simulink model "dx300_boom_hyd"  (R2026b)
settings: Solver=daessc  StopTime=10  AbsTol=1e-3  EnableMultiTasking=on
InitFcn:
  | here='/home/ahmed/ahmed/dx300-sim/matlab/lab08a'; run(fullfile(here,'dx300_params_lab08a.m')); load(fullfile(here,'stage2_mass.mat')); J_cm = P.m_boom*P.L_boom^2/12; La=3.1; phi_rel=deg2rad(-90); m_Dpt=340; m_armpt=1050+220; m_tippt=1120+1.27*1800;
  | S1 = load(fullfile(here,'stage1_kin.mat'),'th','r'); th_tab = S1.th(:)';  r_tab = S1.r(:)';  % moment arm r(theta), m (from ESTIMATED pins)
  | % --- Stage 4 hydraulics ---
  | A_cap = P.n_cyl*pi/4*P.bore^2;                 % OFFICIAL-derived [m^2] combined cap area of 2 cylinders
  | A_ann = P.n_cyl*pi/4*(P.bore^2-P.rod^2);       % OFFICIAL-derived [m^2] combined annulus area
  | rho_oil = 870;      % kg/m^3  ESTIMATED (typical mineral hydraulic oil)
  | beta_oil = 1.5e9;   % Pa      ESTIMATED (typical effective bulk modulus)
  | nu_oil = 46e-6;     % m^2/s   ESTIMATED (ISO VG46-ish, ~46 cSt)
  | A_valve_max = 3e-4; % m^2     ESTIMATED (main spool / relief max area)
  | dS_max = 5e-3;      % m       ESTIMATED (spool stroke)
  | p_range_relief = 5e5; % Pa    ESTIMATED (relief opening range)
  | V_dead = 1e-3;      % m^3     ESTIMATED (dead volume per chamber incl. hose/gallery, both cylinders)
  | % static holding pressure at th_min (analytic gravity torque as in stage3_validate) -> consistent initial cap pressure
  | q0_ = P.th_min; pts_ = [P.L_boom 0; P.L_boom+0.5*La*cos(phi_rel) 0.5*La*sin(phi_rel); P.L_boom+La*cos(phi_rel) La*sin(phi_rel)];
  | tau_g0 = P.m_boom*9.81*Lc0*cos(q0_) + 9.81*([m_Dpt m_armpt m_tippt]*(pts_(:,1)*cos(q0_)-pts_(:,2)*sin(q0_)));   % N m
  | p0_cap = tau_g0/(r_tab(1)*A_cap) + 101325;   % Pa abs
  | spool_t = 1.0;      % s       spool step time (design choice)
values from neighbouring files (symbols this model uses):
  m = dst    [build_stage4.m]    (also in stage2_mass.m = P.m_boom; stage3_validate.m = 'dx300_boom_mb'; stage4_run.m = 'dx300_boom_hyd')
  N = 2^nextpow2(4*numel(pd))    [stage5_damping.m]
  s = get_param([m '/theta_cmd'],'PortHandles')    [stage3_validate.m]    (also in stage4_run.m = Ft.Time > 3)
  Y = abs(fft(pd.*hann(numel(pd)), N))    [stage5_damping.m]
undefined symbols (not defined in the file or in its folder): P, X, Z
libraries: fl_lib x16, nesl_utility x12, sm_lib x11, SimscapeFluids_lib x3, simulink x1
settings Model: Creator=ahmed  LastModifiedBy=ahmed
settings SolverCC: AutoScaleAbsTol=off
settings DataIOCC: LimitDataPoints=on  MaxDataPoints=10000
settings OptimizationCC: LifeSpan=inf  ReuseModelBlockBuffer=off
settings DebuggingCC: AllowSymbolicDim=off  ArithmeticOperatorsInVariantConditions=warning  SFExecutionAtInitializationDiag=none  SFNoUnconditionalDefaultTransitionDiag=warning  SFUnexpectedBacktrackingDiag=warning  SubsystemReferenceDiagnosticForUnitTest=warning
settings SFSimCC: CustomCodeUndefinedFunction=UseInterfaceOnly  SimUseLocalCustomCode=off
settings RTWCC: DLArmComputeVersion=19.05  RTWUseLocalCustomCode=off
settings CodeAppCC: StateflowObjectComments=on
settings GRTTargetCC: TargetLangStandard=C89/C90 (ANSI)
settings ConfigComp: CovExternalEMLEnable=off  CovSFcnEnable=off  CovSaveCumulativeToWorkspaceVar=on  CovSaveSingleToWorkspaceVar=on
settings SimscapeCC: SimscapeLogType=all  SimscapeUseEnergyAccounting=off

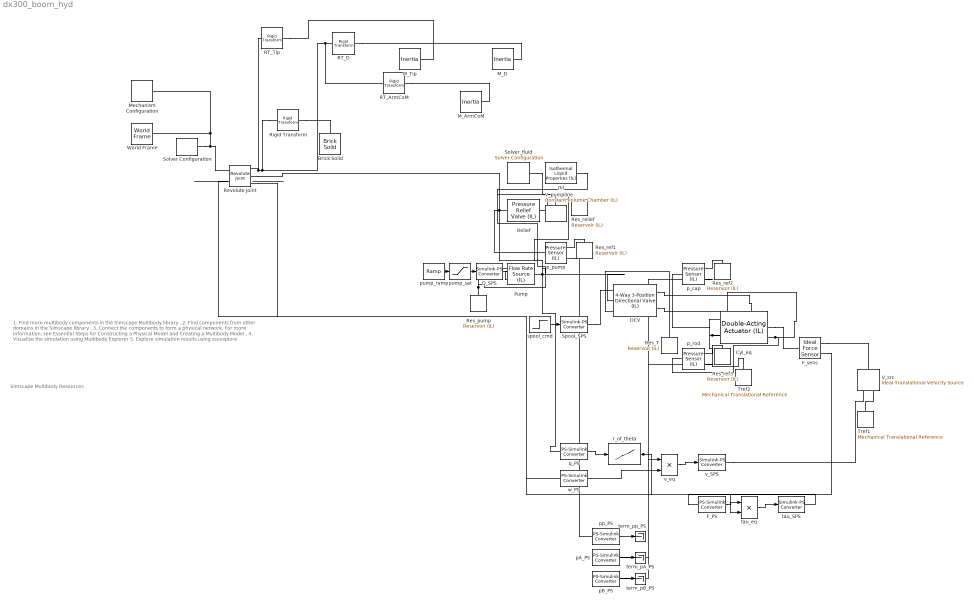
== system dx300_boom_hyd ==
  note: 1. Find more multibody components in the Simscape Multibody library .
      | 2. Find components from other domains in the Simscape library .
      | 3. Connect the components to form a physical network.
      | For more information, see Essential Steps for Constructing a Physical Model and Creating a Multibody Model .
      | 4. Visualize the simulation using Multibody Explorer
      | 5. Explore simulation results using sscexplore
  note: Simscape Multibody Resources
  Brick Solid : sm_lib/Body Elements/Brick Solid  BrickDimensions=[P.L_boom 0.5 0.5]  BrickDimensionsUnits=m  ExportEntireGeometry=off  InertiaType=CalculateFromGeometry  BasedOnType=Mass  Density=1000  DensityUnits=kg/m^3  Mass=2330  MassUnits=kg  CenterOfMass=[0 0 0]  CenterOfMassUnits=m  MomentsOfInertia=[1 1 1]  MomentsOfInertiaUnits=kg*m^2  ProductsOfInertia=[0 0 0]  ProductsOfInertiaUnits=kg*m^2  GraphicType=FromGeometry  MarkerShape=Sphere  MarkerSize=10  GraphicVisPropType=SimpleVisualProperties  GraphicDiffuseColor=[0.5 0.5 0.5]  GraphicOpacity=1.0  GraphicSpecularColor=[0.5 0.5 0.5 1.0]  GraphicAmbientColor=[0.15 0.15 0.15 1.0]  GraphicEmissiveColor=[0.0 0.0 0.0 1.0]  GraphicShininess=75  DoExposeReferenceFrame=on  SerializedFrames=<Frames/>
  Cyl_eq : SimscapeFluids_lib/Isothermal Liquid/Actuators/Double-Acting Actuator (IL)  single_fluid=true  mech_orientation=foundation.enum.MechOrientationTranslational.Positive  piston_area_A=A_cap m^2  piston_area_B=A_ann m^2  stroke=P.stroke m  dead_volume_A=V_dead m^3  dead_volume_B=V_dead m^3  pressure_spec=foundation.enum.pressure_spec.atmospheric  environment_pressure=0.101325 MPa  hardstop_model=simscape.enum.hardstop.smooth  stiff_coeff=1e10 N/m  damping_coeff=150 N*s/m  transition=0.1 mm  coeff_rest=0.7  v_tol=0.001 m/s  f_tol=0.001 N  cushion_A_spec=false  area_plunger_A=1e-4 m^2  length_plunger_A=1e-3 m  area_cushion_orifice_A=1e-6 m^2  area_leak_plunger_A=1e-7 m^2  p_crack_differential_A=0.01 MPa  press_max_differential_A=0.1 MPa  check_valve_area_max_A=1e-4 m^2  check_valve_area_leak_A=1e-10 m^2  smoothing_factor_A=0.01  cushion_B_spec=false  area_plunger_B=1e-4 m^2  length_plunger_B=1e-3 m  area_cushion_orifice_B=1e-6 m^2  area_leak_plunger_B=1e-7 m^2  p_crack_differential_B=0.01 MPa  press_max_differential_B=0.1 MPa  check_valve_area_max_B=1e-4 m^2  check_valve_area_leak_B=1e-10 m^2  smoothing_factor_B=0.01  friction_spec=false  breakaway_Coulomb_ratio=1.2  breakaway_velocity=0.1 m/s  preload_force=20 N  Coulomb_coeff=1e-6 N/Pa  viscous_coeff=100 N*s/m  leakage_spec=false  clearance=1e-4 m  piston_length=0.01 m  displacement_spec=foundation.enum.DisplacementSpec.Calculate  x0=0 m  dynamic_compressibility=true  p0_A=p0_cap Pa  p0_B=0.101325 MPa  p_nominal_A=0.101325 MPa  p_nominal_B=0.101325 MPa
  DCV : SimscapeFluids_lib/Isothermal Liquid/Valves & Orifices/Directional Control Valves/4-Way 3-Position Directional Valve (IL)  open_orifices_pos=fluids.isothermal_liquid.valves_orifices.directional_control_valves.enum.directional_valve_open_orifices_pos_neg.PA_BT  open_orifices_neu=fluids.isothermal_liquid.valves_orifices.directional_control_valves.enum.directional_valve_open_orifices_neutral.all_closed  open_orifices_neg=fluids.isothermal_liquid.valves_orifices.directional_control_valves.enum.directional_valve_open_orifices_pos_neg.PB_AT  neutral_assert_action=simscape.enum.assert.action.warn  area_spec=fluids.isothermal_liquid.valves_orifices.directional_control_valves.enum.directional_valve_area_spec.identical  valve_spec=fluids.isothermal_liquid.valves_orifices.directional_control_valves.enum.directional_valve_spec.linear  del_S_max=dS_max m  area_max=A_valve_max m^2  del_S_TLU=[0, .00125, .0025, .00375, .005] m  valve_area_TLU=[1e-10, 1e-05, 4e-05, 6e-05, .0001] m^2  del_S_vol_flow_TLU=[0, .00125, .0025, .00375, .005] m  p_diff_TLU=[-.1, .3, .5, .7] MPa  vol_flow_TLU=[-1e-08, 2.2e-08, 2.8e-08, 3.4e-08; -9e-06, .00015, .0002, .00024; -.00036, .00063, .00081, .00096; -.00054, .00094, .0012, .0014; -.00091, .0016, .002, .0024] m^3/s  p_diff_TLU_const=[-.1, .3, .5, .7] MPa  vol_flow_TLU_const=[-.0009, .0016, .002, .0024] m^3/s  area_const=1e-4 m^2  area_leak=1e-10 m^2  area=inf m^2  Cd=0.64  Re_c=150  smoothing_factor=0.01  pressure_recovery=false  S_max_PA=7.5e-3 m  del_S_max_PA=0.005 m  area_max_PA=1e-4 m^2  del_S_TLU_PA=[0, .00125, .0025, .00375, .005] m  valve_area_TLU_PA=[1e-10, 1e-05, 4e-05, 6e-05, .0001] m^2  del_S_vol_flow_TLU_PA=[0, .00125, .0025, .00375, .005] m  p_diff_TLU_PA=[-.1, .3, .5, .7] MPa  vol_flow_TLU_PA=[-1e-08, 2.2e-08, 2.8e-08, 3.4e-08; -9e-06, .00015, .0002, .00024; -.00036, .00063, .00081, .00096; -.00054, .00094, .0012, .0014; -.00091, .0016, .002, .0024] m^3/s  area_const_PA=1e-4 m^2  p_diff_TLU_const_PA=[-.1, .3, .5, .7] MPa  vol_flow_TLU_const_PA=[-.0009, .0016, .002, .0024] m^3/s  S_max_PB=-7.5e-3 m  del_S_max_PB=0.005 m  area_max_PB=1e-4 m^2  del_S_TLU_PB=[0, .00125, .0025, .00375, .005] m  valve_area_TLU_PB=[1e-10, 1e-05, 4e-05, 6e-05, .0001] m^2  del_S_vol_flow_TLU_PB=[0, .00125, .0025, .00375, .005] m  p_diff_TLU_PB=[-.1, .3, .5, .7] MPa  vol_flow_TLU_PB=[-1e-08, 2.2e-08, 2.8e-08, 3.4e-08; -9e-06, .00015, .0002, .00024; -.00036, .00063, .00081, .00096; -.00054, .00094, .0012, .0014; -.00091, .0016, .002, .0024] m^3/s  area_const_PB=1e-4 m^2  p_diff_TLU_const_PB=[-.1, .3, .5, .7] MPa  vol_flow_TLU_const_PB=[-.0009, .0016, .002, .0024] m^3/s  S_max_AB=7.5e-3 m  del_S_max_AB=0.005 m  area_max_AB=1e-4 m^2  del_S_TLU_AB=[0, .00125, .0025, .00375, .005] m  valve_area_TLU_AB=[1e-10, 1e-05, 4e-05, 6e-05, .0001] m^2  del_S_vol_flow_TLU_AB=[0, .00125, .0025, .00375, .005] m  p_diff_TLU_AB=[-.1, .3, .5, .7] MPa  vol_flow_TLU_AB=[-1e-08, 2.2e-08, 2.8e-08, 3.4e-08; -9e-06, .00015, .0002, .00024; -.00036, .00063, .00081, .00096; -.00054, .00094, .0012, .0014; -.00091, .0016, .002, .0024] m^3/s  area_const_AB=1e-4 m^2  p_diff_TLU_const_AB=[-.1, .3, .5, .7] MPa  vol_flow_TLU_const_AB=[-.0009, .0016, .002, .0024] m^3/s  S_max_AT=-7.5e-3 m  del_S_max_AT=0.005 m  area_max_AT=1e-4 m^2  del_S_TLU_AT=[0, .00125, .0025, .00375, .005] m  valve_area_TLU_AT=[1e-10, 1e-05, 4e-05, 6e-05, .0001] m^2  del_S_vol_flow_TLU_AT=[0, .00125, .0025, .00375, .005] m  p_diff_TLU_AT=[-.1, .3, .5, .7] MPa  vol_flow_TLU_AT=[-1e-08, 2.2e-08, 2.8e-08, 3.4e-08; -9e-06, .00015, .0002, .00024; -.00036, .00063, .00081, .00096; -.00054, .00094, .0012, .0014; -.00091, .0016, .002, .0024] m^3/s  area_const_AT=1e-4 m^2  p_diff_TLU_const_AT=[-.1, .3, .5, .7] MPa  vol_flow_TLU_const_AT=[-.0009, .0016, .002, .0024] m^3/s  S_max_BT=7.5e-3 m  del_S_max_BT=0.005 m  area_max_BT=1e-4 m^2  del_S_TLU_BT=[0, .00125, .0025, .00375, .005] m  valve_area_TLU_BT=[1e-10, 1e-05, 4e-05, 6e-05, .0001] m^2  del_S_vol_flow_TLU_BT=[0, .00125, .0025, .00375, .005] m  p_diff_TLU_BT=[-.1, .3, .5, .7] MPa  vol_flow_TLU_BT=[-1e-08, 2.2e-08, 2.8e-08, 3.4e-08; -9e-06, .00015, .0002, .00024; -.00036, .00063, .00081, .00096; -.00054, .00094, .0012, .0014; -.00091, .0016, .002, .0024] m^3/s  area_const_BT=1e-4 m^2  p_diff_TLU_const_BT=[-.1, .3, .5, .7] MPa  vol_flow_TLU_const_BT=[-.0009, .0016, .002, .0024] m^3/s  S_max_PT=0 m  del_S_max_PT=0.005 m  area_max_PT=1e-4 m^2  del_S_TLU_PT=[0, .00125, .0025, .00375, .005] m  valve_area_TLU_PT=[1e-10, 1e-05, 4e-05, 6e-05, .0001] m^2  del_S_vol_flow_TLU_PT=[0, .00125, .0025, .00375, .005] m  p_diff_TLU_PT=[-.1, .3, .5, .7] MPa  vol_flow_TLU_PT=[-1e-08, 2.2e-08, 2.8e-08, 3.4e-08; -9e-06, .00015, .0002, .00024; -.00036, .00063, .00081, .00096; -.00054, .00094, .0012, .0014; -.00091, .0016, .002, .0024] m^3/s
  F_PS : nesl_utility/PS-Simulink Converter  PhysicalDomain=network_engine_domain  SubClassName=ps_output  LeftPortType=input  RightPortType=output  PseudoPeriodic=off  Frequencies=[]  VectorFormat=inherit  Unit=N  AffineConversion=off
  F_sens : fl_lib/Mechanical/Mechanical Sensors/Ideal Force Sensor
  M_ArmCoM : sm_lib/Body Elements/Inertia  InertiaType=PointMass  Mass=m_armpt  MassUnits=kg  CenterOfMass=[0 0 0]  CenterOfMassUnits=m  MomentsOfInertia=[1 1 1]  MomentsOfInertiaUnits=kg*m^2  ProductsOfInertia=[0 0 0]  ProductsOfInertiaUnits=kg*m^2  GraphicType=Marker  MarkerShape=Inertia  MarkerSize=20  GraphicVisPropType=SimpleVisualProperties  GraphicDiffuseColor=[0.5 0.5 0.5]  GraphicOpacity=1  GraphicSpecularColor=[0.5 0.5 0.5 1.0]  GraphicAmbientColor=[0.15 0.15 0.15 1.0]  GraphicEmissiveColor=[0.0 0.0 0.0 1.0]  GraphicShininess=75
  M_D : sm_lib/Body Elements/Inertia  InertiaType=PointMass  Mass=m_Dpt  MassUnits=kg  CenterOfMass=[0 0 0]  CenterOfMassUnits=m  MomentsOfInertia=[1 1 1]  MomentsOfInertiaUnits=kg*m^2  ProductsOfInertia=[0 0 0]  ProductsOfInertiaUnits=kg*m^2  GraphicType=Marker  MarkerShape=Inertia  MarkerSize=20  GraphicVisPropType=SimpleVisualProperties  GraphicDiffuseColor=[0.5 0.5 0.5]  GraphicOpacity=1  GraphicSpecularColor=[0.5 0.5 0.5 1.0]  GraphicAmbientColor=[0.15 0.15 0.15 1.0]  GraphicEmissiveColor=[0.0 0.0 0.0 1.0]  GraphicShininess=75
  M_Tip : sm_lib/Body Elements/Inertia  InertiaType=PointMass  Mass=m_tippt  MassUnits=kg  CenterOfMass=[0 0 0]  CenterOfMassUnits=m  MomentsOfInertia=[1 1 1]  MomentsOfInertiaUnits=kg*m^2  ProductsOfInertia=[0 0 0]  ProductsOfInertiaUnits=kg*m^2  GraphicType=Marker  MarkerShape=Inertia  MarkerSize=20  GraphicVisPropType=SimpleVisualProperties  GraphicDiffuseColor=[0.5 0.5 0.5]  GraphicOpacity=1  GraphicSpecularColor=[0.5 0.5 0.5 1.0]  GraphicAmbientColor=[0.15 0.15 0.15 1.0]  GraphicEmissiveColor=[0.0 0.0 0.0 1.0]  GraphicShininess=75
  Mechanism Configuration : sm_lib/Utilities/Mechanism Configuration  UniformGravity=Constant  GravityVector=[0 -9.81 0]  GravityVectorUnits=m/s^2  LinearizationDelta=0.001  JointModeTransitionNonlinearIterations=2
  Oil : fl_lib/Isothermal Liquid/Utilities/Isothermal Liquid Properties (IL)  rho_L_atm=rho_oil kg/m^3  bulk_modulus_model=foundation.enum.bulk_modulus_model.const  beta_gain=6  beta_L_atm=beta_oil Pa  nu_atm=nu_oil m^2/s  p_atm=0.101325 MPa  p_min=1 Pa  properties_range_check=simscape.enum.assert.action.error  air_fraction=0.005  polytropic_index=1.0  rho_g_atm=1.225 kg/m^3  air_dissolution_model=false  p_crit=3 MPa
  Pump : fl_lib/Isothermal Liquid/Sources/Flow Rate Source (IL)  source_type=foundation.enum.constant_controlled.controlled  flow_type=foundation.enum.mass_volumetric_flow.volumetric  mass_flow=0 kg/s  volumetric_flow=0 m^3/s
  Q_SPS : nesl_utility/Simulink-PS Converter  PhysicalDomain=network_engine_domain  SubClassName=ps_input  LeftPortType=input  RightPortType=output  PseudoPeriodic=off  Frequencies=[]  NoiseDistribution=none  NoiseParameters=[]  Unit=m^3/s  AffineConversion=off  FilteringAndDerivatives=filter  SimscapeFilterOrder=2  InputFilterTimeConstant=0.001  UdotUserProvided=0
  RT_ArmCoM : sm_lib/Frames and Transforms/Rigid Transform  RotationMethod=None  FollAlignAxisA=+X  BaseAlignAxisA=+Y  FollAlignAxisB=+Y  BaseAlignAxisB=+Z  RotationStandardAxis=+Z  RotationAngle=0  RotationAngleUnits=deg  RotationArbitraryAxis=[0 0 1]  RotationSequenceAxes=FollowerAxes  RotationSequence=XYX  RotationSequenceAngles=[0 0 0]  RotationSequenceAnglesUnits=deg  RotationMatrix=[1 0 0;0 1 0;0 0 1]  Quaternion=[1 0 0 0]  TranslationMethod=Cartesian  TranslationCartesianOffset=[P.L_boom+0.5*La*cos(phi_rel) 0.5*La*sin(phi_rel) 0]  TranslationCartesianOffsetUnits=m  TranslationStandardAxis=+Z  TranslationStandardOffset=0  TranslationStandardOffsetUnits=m  TranslationROffset=0  TranslationROffsetUnits=m  TranslationThetaOffset=0  TranslationThetaOffsetUnits=deg  TranslationZOffset=0  TranslationZOffsetUnits=m
  RT_D : sm_lib/Frames and Transforms/Rigid Transform  RotationMethod=None  FollAlignAxisA=+X  BaseAlignAxisA=+Y  FollAlignAxisB=+Y  BaseAlignAxisB=+Z  RotationStandardAxis=+Z  RotationAngle=0  RotationAngleUnits=deg  RotationArbitraryAxis=[0 0 1]  RotationSequenceAxes=FollowerAxes  RotationSequence=XYX  RotationSequenceAngles=[0 0 0]  RotationSequenceAnglesUnits=deg  RotationMatrix=[1 0 0;0 1 0;0 0 1]  Quaternion=[1 0 0 0]  TranslationMethod=Cartesian  TranslationCartesianOffset=[P.L_boom 0 0]  TranslationCartesianOffsetUnits=m  TranslationStandardAxis=+Z  TranslationStandardOffset=0  TranslationStandardOffsetUnits=m  TranslationROffset=0  TranslationROffsetUnits=m  TranslationThetaOffset=0  TranslationThetaOffsetUnits=deg  TranslationZOffset=0  TranslationZOffsetUnits=m
  RT_Tip : sm_lib/Frames and Transforms/Rigid Transform  RotationMethod=None  FollAlignAxisA=+X  BaseAlignAxisA=+Y  FollAlignAxisB=+Y  BaseAlignAxisB=+Z  RotationStandardAxis=+Z  RotationAngle=0  RotationAngleUnits=deg  RotationArbitraryAxis=[0 0 1]  RotationSequenceAxes=FollowerAxes  RotationSequence=XYX  RotationSequenceAngles=[0 0 0]  RotationSequenceAnglesUnits=deg  RotationMatrix=[1 0 0;0 1 0;0 0 1]  Quaternion=[1 0 0 0]  TranslationMethod=Cartesian  TranslationCartesianOffset=[P.L_boom+La*cos(phi_rel) La*sin(phi_rel) 0]  TranslationCartesianOffsetUnits=m  TranslationStandardAxis=+Z  TranslationStandardOffset=0  TranslationStandardOffsetUnits=m  TranslationROffset=0  TranslationROffsetUnits=m  TranslationThetaOffset=0  TranslationThetaOffsetUnits=deg  TranslationZOffset=0  TranslationZOffsetUnits=m
  Relief : SimscapeFluids_lib/Isothermal Liquid/Valves & Orifices/Pressure Control Valves/Pressure Relief Valve (IL)  set_pressure_spec=foundation.enum.constant_controlled.constant  opening_spec=fluids.isothermal_liquid.valves_orifices.enum.PressureOpeningSpec.Linear  pressure_spec=fluids.isothermal_liquid.valves_orifices.enum.pressure_control_spec.pA  p_set_gauge=P.p_relief Pa  p_set_differential=0 MPa  p_range=p_range_relief Pa  area_max=A_valve_max m^2  area_leak=1e-10 m^2  p_diff_TLU=[0.2 : 0.2 : 1.2] MPa  p_gauge_TLU=[0.2 : 0.2 : 1.2] MPa  valve_area_TLU=[1e-10, 2e-06, 4e-06, 6e-06, 8e-06, 1e-05] m^2  vol_flow_TLU=[1e-09, 3.6e-05, 8.9e-05, .00015, .00023, .00031] m^3/s  area=inf m^2  Cd=0.64  Re_c=150  smoothing_factor=0.01  pressure_recovery=false  opening_dynamics=false  tau=0.1 s
  Res_T : fl_lib/Isothermal Liquid/Elements/Reservoir (IL)  pressure_input=false  pressure_spec=foundation.enum.pressure_spec.atmospheric  reservoir_pressure=0.101325 MPa
  Res_pump : fl_lib/Isothermal Liquid/Elements/Reservoir (IL)  pressure_input=false  pressure_spec=foundation.enum.pressure_spec.atmospheric  reservoir_pressure=0.101325 MPa
  Res_ref1 : fl_lib/Isothermal Liquid/Elements/Reservoir (IL)  pressure_input=false  pressure_spec=foundation.enum.pressure_spec.atmospheric  reservoir_pressure=0.101325 MPa
  Res_ref2 : fl_lib/Isothermal Liquid/Elements/Reservoir (IL)  pressure_input=false  pressure_spec=foundation.enum.pressure_spec.atmospheric  reservoir_pressure=0.101325 MPa
  Res_ref3 : fl_lib/Isothermal Liquid/Elements/Reservoir (IL)  pressure_input=false  pressure_spec=foundation.enum.pressure_spec.atmospheric  reservoir_pressure=0.101325 MPa
  Res_relief : fl_lib/Isothermal Liquid/Elements/Reservoir (IL)  pressure_input=false  pressure_spec=foundation.enum.pressure_spec.atmospheric  reservoir_pressure=0.101325 MPa
  Revolute Joint : sm_lib/Joints/Revolute Joint  JointMode=Normal  CompositeWrenchDir=FollowerOnBase  CompositeWrenchFrame=BaseFrame  SenseConstraintForce=off  SenseConstraintTorque=off  SenseTotalForce=off  SenseTotalTorque=off  PositionTargetSpecify=on  PositionTargetPriority=High  PositionTargetValue=P.th_min*180/pi  PositionTargetValueUnits=deg  VelocityTargetSpecify=off  VelocityTargetPriority=High  VelocityTargetValue=0  VelocityTargetValueUnits=deg/s  EquilibriumPosition=0  EquilibriumPositionUnits=deg  SpringStiffness=0  SpringStiffnessUnits=N*m/deg  DampingCoefficient=0  DampingCoefficientUnits=N*m/(deg/s)  LowerLimitSpecify=off  LowerLimitBound=-90  LowerLimitBoundUnits=deg  LowerLimitStiffness=1e4  LowerLimitStiffnessUnits=N*m/deg  LowerLimitDamping=10  LowerLimitDampingUnits=N*m/(deg/s)  LowerLimitTransitionRegionWidth=0.1  LowerLimitTransitionRegionWidthUnits=deg  UpperLimitSpecify=off  UpperLimitBound=90  UpperLimitBoundUnits=deg  UpperLimitStiffness=1e4  UpperLimitStiffnessUnits=N*m/deg  UpperLimitDamping=10  UpperLimitDampingUnits=N*m/(deg/s)  UpperLimitTransitionRegionWidth=0.1  UpperLimitTransitionRegionWidthUnits=deg  TorqueActuationMode=InputTorque  MotionActuationMode=ComputedMotion  SensePosition=on  SenseVelocity=on  SenseAcceleration=off  SenseTorqueForce=off  SenseLowerLimitTorqueForce=off  SenseUpperLimitTorqueForce=off
  Rigid Transform : sm_lib/Frames and Transforms/Rigid Transform  RotationMethod=StandardAxis  FollAlignAxisA=+X  BaseAlignAxisA=+Y  FollAlignAxisB=+Y  BaseAlignAxisB=+Z  RotationStandardAxis=+X  RotationAngle=0.0  RotationAngleUnits=deg  RotationArbitraryAxis=[0 0 1]  RotationSequenceAxes=FollowerAxes  RotationSequence=XYX  RotationSequenceAngles=[0 0 0]  RotationSequenceAnglesUnits=deg  RotationMatrix=[1 0 0; 0 1 0; 0 0 1]  Quaternion=[1 0 0 0]  TranslationMethod=StandardAxis  TranslationCartesianOffset=[0 0 0]  TranslationCartesianOffsetUnits=m  TranslationStandardAxis=+X  TranslationStandardOffset=Lc0  TranslationStandardOffsetUnits=m  TranslationROffset=0  TranslationROffsetUnits=m  TranslationThetaOffset=0  TranslationThetaOffsetUnits=deg  TranslationZOffset=0  TranslationZOffsetUnits=m
  Solver Configuration : nesl_utility/Solver Configuration  PhysicalDomain=network_engine_domain  SubClassName=solver  LeftPortType=input  RightPortType=generic  Tones=[]  Harmonics=[]  SimulateNoise=off  Profile=off  UseLocalSampling=off  EnableSwitchedLinearOptims=on  FrequencyDomain=off  UseCCode=off  RelTol=0.001  AbsTol=1e-06  MinStep=1e-09  ToWorkspace=off  RevertToSquareIcSolve=off  NumHomotopyIterations=100  PhasorMode=off  PhasorModeNumHarmonics=1  ConsistencySolver=NEWTON_XTOL_AFTER_FTOL  CanonicalOrdering=UNORDERED  OptimizeIntermediates=UNOPTIMIZED  MulticoreSolverChoice=BACKWARD_EULER  IndexReductionMethod=DerivativeReplacement  DoDC=off  ResidualTolerance=1e-09  ConsistencyTolSource=GLOBAL  ConsistencyAbsTol=0.001  ConsistencyRelTol=0.001  ConsistencyTolFactor=0.001  UseLocalSolver=off  LocalSolverChoice=NE_BACKWARD_EULER_ADVANCER  ResolveIndetEquations=on  FunctionEvalNumThread=1  LocalSolverSampleTime=0.001  DoFixedCost=off  MaxNonlinIter=3  MaxModeIter=2  ComputeImpulses=off  ImpulseIterations=2  LinearAlgebra=Sparse  LinearAlgebraNumThread=0  EquationFormulation=NE_TIME_EF  DelaysMemoryBudget=1024  AutomaticFiltering=on  FilteringTimeConstant=0.001  PartitionStorageMethod=AS_NEEDED  PartitionMemoryBudget=1024  PartitionMethod=FAST  MultibodyUseLocalSolver=off  MultibodyLocalSolverChoice=ODE1  MultibodyLocalSolverSampleTime=0.001
  Solver_fluid : nesl_utility/Solver Configuration  PhysicalDomain=network_engine_domain  SubClassName=solver  LeftPortType=input  RightPortType=generic  Tones=[]  Harmonics=[]  SimulateNoise=off  Profile=off  UseLocalSampling=off  EnableSwitchedLinearOptims=on  FrequencyDomain=off  UseCCode=off  RelTol=0.001  AbsTol=1e-06  MinStep=1e-09  ToWorkspace=off  RevertToSquareIcSolve=off  NumHomotopyIterations=100  PhasorMode=off  PhasorModeNumHarmonics=1  ConsistencySolver=NEWTON_XTOL_AFTER_FTOL  CanonicalOrdering=UNORDERED  OptimizeIntermediates=UNOPTIMIZED  MulticoreSolverChoice=BACKWARD_EULER  IndexReductionMethod=DerivativeReplacement  DoDC=off  ResidualTolerance=1e-09  ConsistencyTolSource=GLOBAL  ConsistencyAbsTol=0.001  ConsistencyRelTol=0.001  ConsistencyTolFactor=0.001  UseLocalSolver=off  LocalSolverChoice=NE_BACKWARD_EULER_ADVANCER  ResolveIndetEquations=on  FunctionEvalNumThread=1  LocalSolverSampleTime=0.001  DoFixedCost=off  MaxNonlinIter=3  MaxModeIter=2  ComputeImpulses=off  ImpulseIterations=2  LinearAlgebra=Sparse  LinearAlgebraNumThread=0  EquationFormulation=NE_TIME_EF  DelaysMemoryBudget=1024  AutomaticFiltering=on  FilteringTimeConstant=0.001  PartitionStorageMethod=AS_NEEDED  PartitionMemoryBudget=1024  PartitionMethod=FAST  MultibodyUseLocalSolver=off  MultibodyLocalSolverChoice=ODE1  MultibodyLocalSolverSampleTime=0.001
  Spool_SPS : nesl_utility/Simulink-PS Converter  PhysicalDomain=network_engine_domain  SubClassName=ps_input  LeftPortType=input  RightPortType=output  PseudoPeriodic=off  Frequencies=[]  NoiseDistribution=none  NoiseParameters=[]  Unit=m  AffineConversion=off  FilteringAndDerivatives=filter  SimscapeFilterOrder=2  InputFilterTimeConstant=0.001  UdotUserProvided=0
  Tref1 : fl_lib/Mechanical/Translational Elements/Mechanical Translational Reference
  Tref2 : fl_lib/Mechanical/Translational Elements/Mechanical Translational Reference
  V_pumpline : fl_lib/Isothermal Liquid/Elements/Constant Volume Chamber (IL)  volume=2e-3 m^3  p_I_specify=off  p_I_priority=High  p_I=0.101325 MPa  p_I_nominal_specify=off  p_I_nominal_value=1  p_I_nominal_unit=MPa
  V_src : fl_lib/Mechanical/Mechanical Sources/Ideal Translational Velocity Source
  World Frame : sm_lib/Frames and Transforms/World Frame
  pA_PS : nesl_utility/PS-Simulink Converter  PhysicalDomain=network_engine_domain  SubClassName=ps_output  LeftPortType=input  RightPortType=output  PseudoPeriodic=off  Frequencies=[]  VectorFormat=inherit  Unit=Pa  AffineConversion=off
  pB_PS : nesl_utility/PS-Simulink Converter  PhysicalDomain=network_engine_domain  SubClassName=ps_output  LeftPortType=input  RightPortType=output  PseudoPeriodic=off  Frequencies=[]  VectorFormat=inherit  Unit=Pa  AffineConversion=off
  p_cap : fl_lib/Isothermal Liquid/Sensors/Pressure Sensor (IL)  pressure_measure=foundation.enum.pressure_measure.difference
  p_pump : fl_lib/Isothermal Liquid/Sensors/Pressure Sensor (IL)  pressure_measure=foundation.enum.pressure_measure.difference
  p_rod : fl_lib/Isothermal Liquid/Sensors/Pressure Sensor (IL)  pressure_measure=foundation.enum.pressure_measure.difference
  pp_PS : nesl_utility/PS-Simulink Converter  PhysicalDomain=network_engine_domain  SubClassName=ps_output  LeftPortType=input  RightPortType=output  PseudoPeriodic=off  Frequencies=[]  VectorFormat=inherit  Unit=Pa  AffineConversion=off
  pump_ramp : simulink/Sources/Ramp  slope=P.Q_pump/0.2  start=0  InitialOutput=0
  pump_sat : Saturate  UpperLimit=P.Q_pump  LowerLimit=0
  q_PS : nesl_utility/PS-Simulink Converter  PhysicalDomain=network_engine_domain  SubClassName=ps_output  LeftPortType=input  RightPortType=output  PseudoPeriodic=off  Frequencies=[]  VectorFormat=inherit  Unit=rad  AffineConversion=off
  r_of_theta : Lookup_n-D  NumberOfTableDimensions=1  BreakpointsForDimension1=th_tab  Table=r_tab  ExtrapMethod=Clip  InternalRulePriority=Speed  RndMeth=Simplest
  spool_cmd : Step  Time=spool_t  FinalValue=dS_max  SampleTime=0
  tau_SPS : nesl_utility/Simulink-PS Converter  PhysicalDomain=network_engine_domain  SubClassName=ps_input  LeftPortType=input  RightPortType=output  PseudoPeriodic=off  Frequencies=[]  NoiseDistribution=none  NoiseParameters=[]  Unit=N*m  AffineConversion=off  FilteringAndDerivatives=filter  SimscapeFilterOrder=2  InputFilterTimeConstant=0.001  UdotUserProvided=0
  tau_eq : Product
  term_pA_PS : Terminator
  term_pB_PS : Terminator
  term_pp_PS : Terminator
  v_SPS : nesl_utility/Simulink-PS Converter  PhysicalDomain=network_engine_domain  SubClassName=ps_input  LeftPortType=input  RightPortType=output  PseudoPeriodic=off  Frequencies=[]  NoiseDistribution=none  NoiseParameters=[]  Unit=m/s  AffineConversion=off  FilteringAndDerivatives=filter  SimscapeFilterOrder=2  InputFilterTimeConstant=0.001  UdotUserProvided=0
  v_eq : Product
  w_PS : nesl_utility/PS-Simulink Converter  PhysicalDomain=network_engine_domain  SubClassName=ps_output  LeftPortType=input  RightPortType=output  PseudoPeriodic=off  Frequencies=[]  VectorFormat=inherit  Unit=rad/s  AffineConversion=off
  wires:
  ? -> ?
  ? -> ?
  q_PS/1 -> r_of_theta/1
  r_of_theta/1 -> v_eq/1, tau_eq/2
  w_PS/1 -> v_eq/2
  v_eq/1 -> v_SPS/1
  F_PS/1 -> tau_eq/1
  tau_eq/1 -> tau_SPS/1
  spool_cmd/1 -> Spool_SPS/1
  pump_ramp/1 -> pump_sat/1
  pump_sat/1 -> Q_SPS/1
  pp_PS/1 -> term_pp_PS/1
  pA_PS/1 -> term_pA_PS/1
  pB_PS/1 -> term_pB_PS/1
  connections:
  Rigid Transform/RConn1 -- Brick Solid/RConn1
  ?
  Rigid Transform/LConn1 -- RT_D/LConn1 -- RT_ArmCoM/LConn1 -- Revolute Joint/RConn1 -- RT_Tip/LConn1
  ?
  Solver Configuration/RConn1 -- World Frame/RConn1 -- Mechanism Configuration/RConn1 -- Revolute Joint/LConn1
  RT_D/RConn1 -- M_D/RConn1
  RT_ArmCoM/RConn1 -- M_ArmCoM/RConn1
  RT_Tip/RConn1 -- M_Tip/RConn1
  Revolute Joint/LConn2 -- tau_SPS/RConn1
  Revolute Joint/RConn2 -- q_PS/LConn1
  Revolute Joint/RConn3 -- w_PS/LConn1
  v_SPS/RConn1 -- V_src/RConn1
  Cyl_eq/RConn2 -- F_sens/LConn1
  F_sens/RConn1 -- V_src/LConn1
  V_src/RConn2 -- Tref1/LConn1
  Cyl_eq/LConn1 -- Tref2/LConn1
  F_sens/RConn2 -- F_PS/LConn1
  Res_pump/LConn1 -- Pump/LConn1 -- Solver_fluid/RConn1
  Q_SPS/RConn1 -- Pump/LConn2
  Pump/RConn1 -- DCV/LConn2 -- V_pumpline/LConn1 -- Oil/RConn1 -- Relief/LConn1 -- p_pump/LConn1
  Relief/RConn1 -- Res_relief/LConn1
  Res_T/LConn1 -- DCV/LConn3
  Cyl_eq/LConn2 -- DCV/RConn1 -- p_cap/LConn1
  Cyl_eq/RConn3 -- DCV/RConn2 -- p_rod/LConn1
  Spool_SPS/RConn1 -- DCV/LConn1
  p_pump/RConn1 -- Res_ref1/LConn1
  p_pump/RConn2 -- pp_PS/LConn1
  p_cap/RConn1 -- Res_ref2/LConn1
  p_cap/RConn2 -- pA_PS/LConn1
  p_rod/RConn1 -- Res_ref3/LConn1
  p_rod/RConn2 -- pB_PS/LConn1
